simulink model "motor_lqr_intro"  (R2025b)
settings: Solver=ode45  StartTime=0.0  StopTime=5  MaxStep=0.01  RelTol=1e-8  AbsTol=1e-10
model workspace (MAT data in the model file):
  A = [-1  10; -1  -10]
  B = [0; 10]
  K = [2.80954174833 1.59211949892]
  Q = [10  0; 0  0.1]
  Ru = 1
  i_ref = 1
  omega_ref = 10
  u_ref = 2
  x_ref = [10; 1]
settings Model: Creator=alosw  LastModifiedBy=alosw

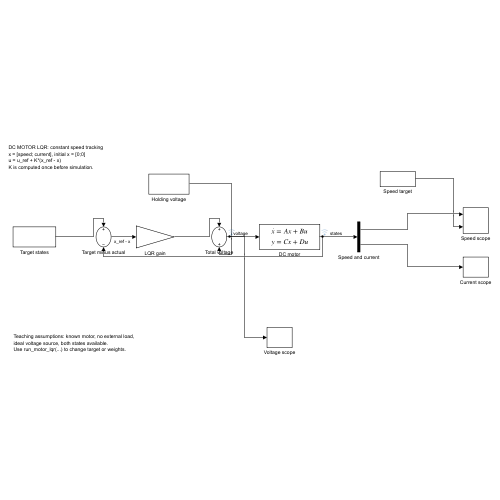
[thumbnail: Simulink's stored preview of the top-level diagram]
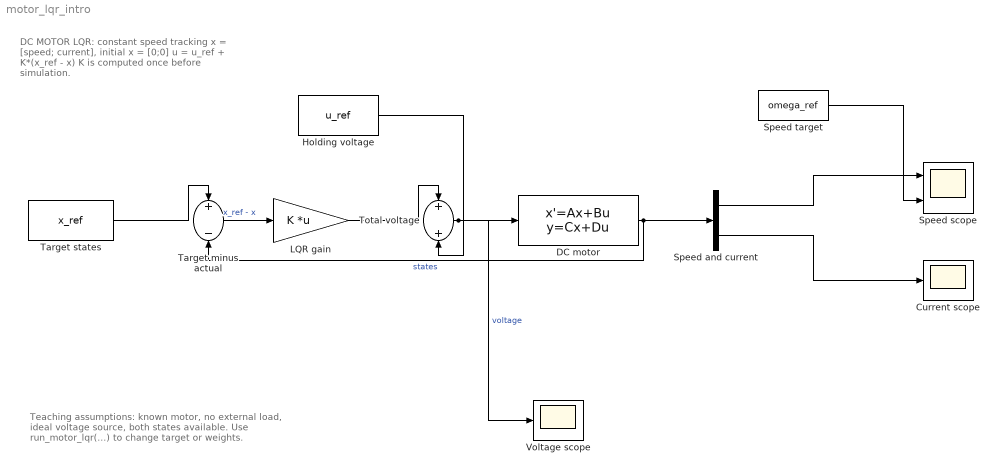
== system motor_lqr_intro ==
  note: DC MOTOR LQR: constant speed tracking
      | x = [speed; current], initial x = [0;0]
      | u = u_ref + K*(x_ref - x)
      | K is computed once before simulation.
  note: Teaching assumptions: known motor, no external load,
      | ideal voltage source, both states available.
      | Use run_motor_lqr(...) to change target or weights.
  Current scope : Scope
  DC motor : StateSpace  A=A  B=B  C=eye(2)  D=zeros(2,1)  InitialCondition=[0;0]
  Holding voltage : Constant  Value=u_ref
  LQR gain : Gain  Gain=K  Multiplication=Matrix(K*u)
  Speed and current : Demux  Outputs=2
  Speed scope : Scope  NumInputPorts=2
  Speed target : Constant  Value=omega_ref
  Target minus actual : Sum  Inputs=+-
  Target states : Constant  Value=x_ref
  Total voltage : Sum
  Voltage scope : Scope
  wires:
  Target states/1 -> Target minus actual/1
  Target minus actual/1 -> LQR gain/1  "x_ref - x"
  LQR gain/1 -> Total voltage/1
  Holding voltage/1 -> Total voltage/2
  Total voltage/1 -> DC motor/1, Voltage scope/1  "voltage"
  DC motor/1 -> Speed and current/1, Target minus actual/2  "states"
  Speed and current/1 -> Speed scope/1
  Speed target/1 -> Speed scope/2
  Speed and current/2 -> Current scope/1
